simulink model "dpsim_rlc_me"  (R2025a)
settings: Solver=ode45  StartTime=0  StopTime=0.10000000000000001  MaxStep=1.0000000000000001e-05  RelTol=1e-9  AbsTol=1e-10
settings Model: Creator=matthiasmees  LastModifiedBy=matthiasmees

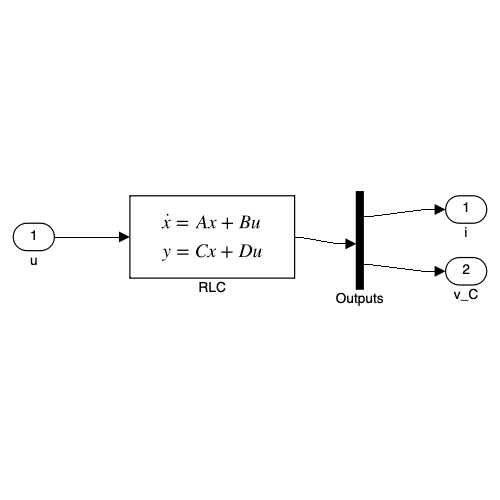
[thumbnail: Simulink's stored preview of the top-level diagram]
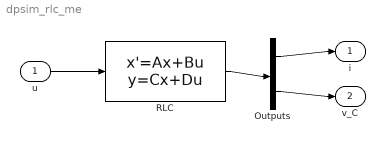
== system dpsim_rlc_me ==
  u : Inport
  Outputs : Demux  Outputs=2
  RLC : StateSpace  A=[-500 -50;10000 0]  B=[50;0]  C=[1 0;0 1]  D=[0;0]  InitialCondition=[0;0]
  i : Outport
  v_C : Outport  Port=2
  wires:
  u/1 -> RLC/1
  RLC/1 -> Outputs/1
  Outputs/1 -> i/1
  Outputs/2 -> v_C/1
